simulink model "SSW3D"  (R2023a)
settings: Solver=ode4  StartTime=0.0  StopTime=viz_Tend  FixedStep=viz_Ts  RelTol=1e-3
undefined symbols (not defined in the file): viz_Ts
libraries: sim3dlib x3, sim3dautolib x2
settings Model: Creator=Tan_Tram  LastModifiedBy=Tan_Tram

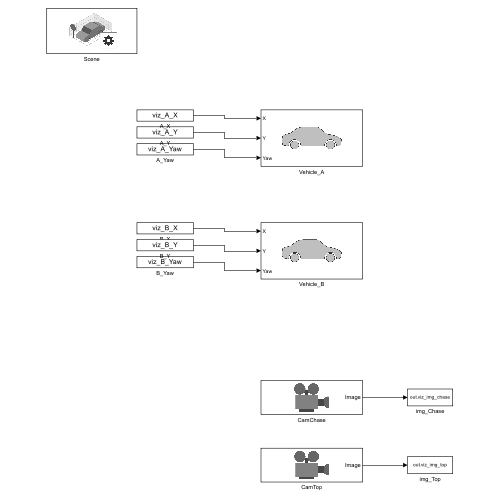
[thumbnail: Simulink's stored preview of the top-level diagram]
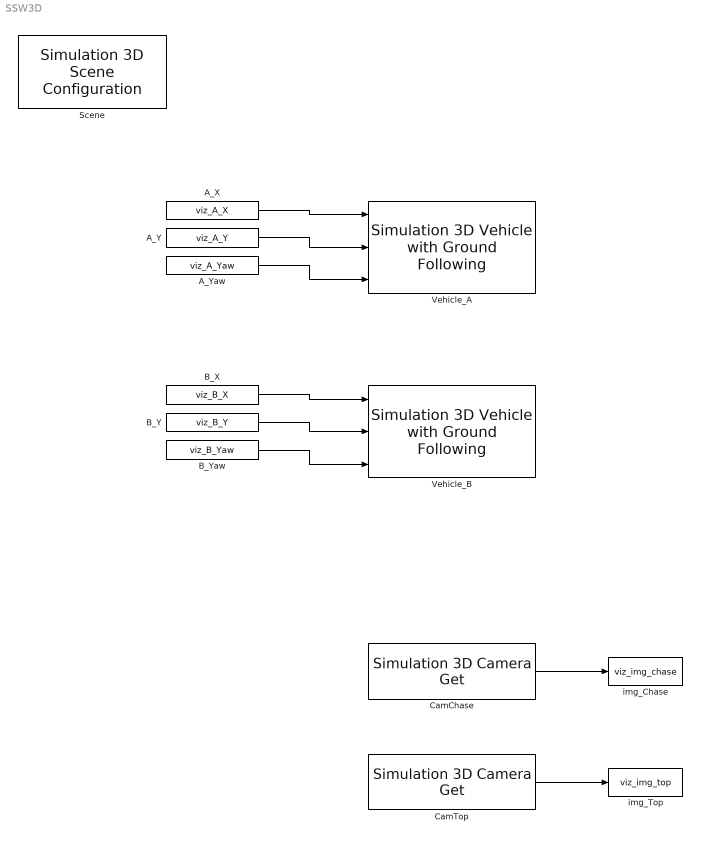
== system SSW3D ==
  A_X : FromWorkspace  VariableName=viz_A_X  SampleTime=viz_Ts  OutputAfterFinalValue=Holding final value
  A_Y : FromWorkspace  VariableName=viz_A_Y  SampleTime=viz_Ts  OutputAfterFinalValue=Holding final value
  A_Yaw : FromWorkspace  VariableName=viz_A_Yaw  SampleTime=viz_Ts  OutputAfterFinalValue=Holding final value
  B_X : FromWorkspace  VariableName=viz_B_X  SampleTime=viz_Ts  OutputAfterFinalValue=Holding final value
  B_Y : FromWorkspace  VariableName=viz_B_Y  SampleTime=viz_Ts  OutputAfterFinalValue=Holding final value
  B_Yaw : FromWorkspace  VariableName=viz_B_Yaw  SampleTime=viz_Ts  OutputAfterFinalValue=Holding final value
  CamChase : sim3dlib/Simulation 3D Camera Get  Priority=1  sensorTag=Sim3dSensor1  sensorId=1  sensorName=CamChase  vehTagList={'Scene Origin', 'VehA', 'VehB'}  vehTag=VehA  mountLoc=Origin  offsetFlag=on  tmountOffset=[-14 0 5]  rmountOffset=[0 12 0]  HorizontalResolution=960  VerticalResolution=540  HorizontalFOV=60  SampleTime=viz_Ts  mountPoint=[0 0 0]  mountOrientation=[0 0 0]  aMode=aMode  ID=1
  CamTop : sim3dlib/Simulation 3D Camera Get  Priority=1  sensorTag=Sim3dSensor2  sensorId=2  sensorName=CamTop  vehTagList={'Scene Origin', 'VehA', 'VehB'}  vehTag=VehA  mountLoc=Origin  offsetFlag=on  tmountOffset=[0 0 35]  rmountOffset=[0 90 0]  HorizontalResolution=960  VerticalResolution=540  HorizontalFOV=60  SampleTime=viz_Ts  mountPoint=[0 0 0]  mountOrientation=[0 0 0]  aMode=aMode  ID=2
  Scene : sim3dlib/Simulation 3D Scene Configuration  Priority=0  ProjectFormat=Default Scenes  SceneDesc=Open surface  ProjectName=C:\Program Files\MATLAB\R2023a\toolbox\shared\sim3d_projects\automotive_project\UE4\WindowsNoEditor\VehicleSimulation.exe  ScenePath=/Game/Maps/HwStrght  EnableOpenDRIVE=off  vehTagList={'Scene Origin'}  vehTag=Scene Origin  OpVisEn=off  Ts=viz_Ts  EnableWindow=on  EnableRemoteAccess=off  EnableWeather=off  SunAltitude=40.0  SunAzimuth=90  clouds=10  wind=1  fog=0  rain=0  EnableGeospatial=off  OriginHeight=200  OriginLatitude=40.744652  OriginLongitude=-73.988864  MapStyle=Aerial  AdditionalAssetIDs=[]  UseAdvancedSunSky=off  SolarTime=11  TimeZone=-5  Day=21  Month=9  Year=2022  UseDaylightSavingTime=on  DSTStartDay=10  DSTStartMonth=3  DSTEndDay=3  DSTEndMonth=11  DSTSwitchHour=2  sensorTag=MainCamera1  sensorId=1  sensorName=MainCamera1  mountLoc=Origin  offsetFlag=off  tmountOffset=[0, 0, 0]  rmountOffset=[0, 0, 0]  HorizontalResolution=1280  VerticalResolution=720  HorizontalFOV=60  mountPoint=[0 0 0]  mountOrientation=[0 0 0]  aMode=aMode  ID=1  GeoTrigger=Inactive
  Vehicle_A : sim3dautolib/Simulation 3D Vehicle with Ground Following  Priority=-1  PassVehMesh=Sedan  MeshPath=/MathWorksAutomotiveContent/Vehicles/Muscle/Meshes/SK_MuscleCar.SK_MuscleCar  TrackWidth=1.9  WheelBase=3  WheelRadius=0.35  VehColor=Red  InitialPos=[0, 0, 0]  InitialRot=[0, 0, 0]  ActorName=VehA  SampleTime=viz_Ts  ActorType=SimulinkVehicle  ID=C  aMode=aMode  ActorTag=VehA  CoordinateScheme=ISO  VehLightsControl=off  HeadlightColor=[ 1, 1, 1 ]  HighBeamIntensity=100000  LowBeamIntensity=60000  HighBeamConeAngle=70  LowBeamConeAngle=70  LeftHeadlightOrientation=[ 0, 0 ]  RightHeadlightOrientation=[ 0, 0 ]  BrakelightIntensity=500  ReverselightIntensity=500  SignallightIntensity=500  SignallightPeriod=1  SignalPulseWidth=50  TransformOutportEnabled=off
  Vehicle_B : sim3dautolib/Simulation 3D Vehicle with Ground Following  Priority=-1  PassVehMesh=Sedan  MeshPath=/MathWorksAutomotiveContent/Vehicles/Muscle/Meshes/SK_MuscleCar.SK_MuscleCar  TrackWidth=1.9  WheelBase=3  WheelRadius=0.35  VehColor=Blue  InitialPos=[0, 0, 0]  InitialRot=[0, 0, 0]  ActorName=VehB  SampleTime=viz_Ts  ActorType=SimulinkVehicle  ID=C  aMode=aMode  ActorTag=VehB  CoordinateScheme=ISO  VehLightsControl=off  HeadlightColor=[ 1, 1, 1 ]  HighBeamIntensity=100000  LowBeamIntensity=60000  HighBeamConeAngle=70  LowBeamConeAngle=70  LeftHeadlightOrientation=[ 0, 0 ]  RightHeadlightOrientation=[ 0, 0 ]  BrakelightIntensity=500  ReverselightIntensity=500  SignallightIntensity=500  SignallightPeriod=1  SignalPulseWidth=50  TransformOutportEnabled=off
  img_Chase : ToWorkspace  VariableName=viz_img_chase  SaveFormat=Timeseries  SampleTime=viz_Ts
  img_Top : ToWorkspace  VariableName=viz_img_top  SaveFormat=Timeseries  SampleTime=viz_Ts
  wires:
  A_X/1 -> Vehicle_A/1
  A_Y/1 -> Vehicle_A/2
  A_Yaw/1 -> Vehicle_A/3
  B_X/1 -> Vehicle_B/1
  B_Y/1 -> Vehicle_B/2
  B_Yaw/1 -> Vehicle_B/3
  CamChase/1 -> img_Chase/1
  CamTop/1 -> img_Top/1
